simulink model "scheme_L2"  (R2021b)
settings: Solver=ode45  StartTime=0.0  StopTime=10.0  MaxStep=0.001  RelTol=1e-6  AbsTol=1e-8
settings Model: Creator=ALIENWARE  LastModifiedBy=ALIENWARE

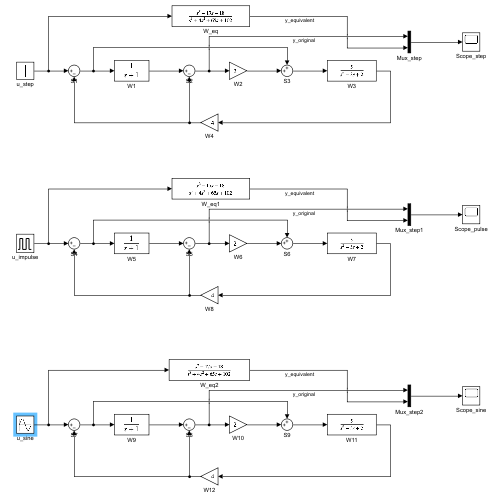
[thumbnail: Simulink's stored preview of the top-level diagram]
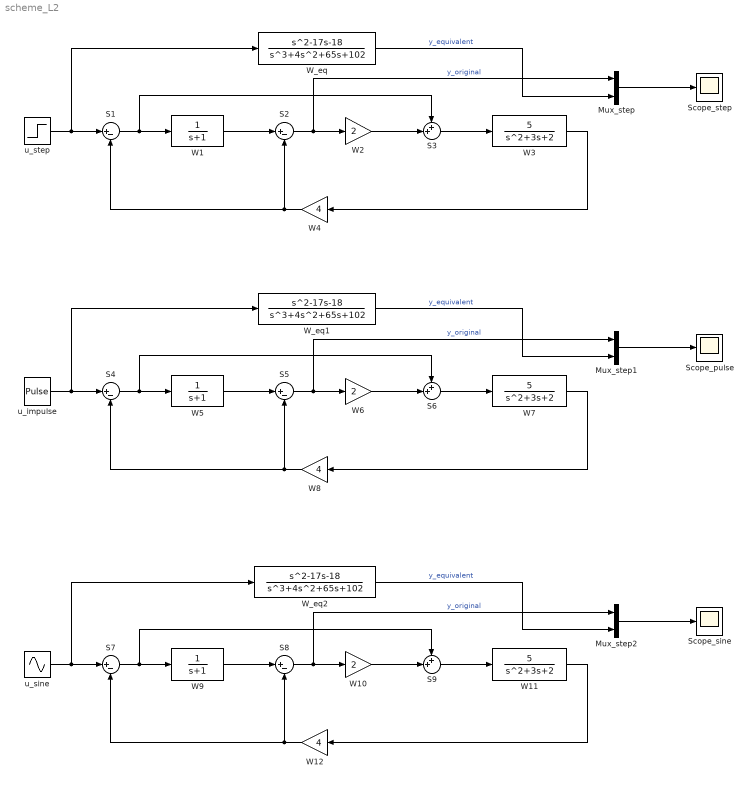
== system scheme_L2 ==
  Mux_step : Mux  Inputs=2
  Mux_step1 : Mux  Inputs=2
  Mux_step2 : Mux  Inputs=2
  S{1..2,4..5,7..8} (6 alike) : Sum  Inputs=|+-
  S3 : Sum  Inputs=++|
  S6 : Sum  Inputs=++|
  S9 : Sum  Inputs=++|
  Scope_pulse : Scope
  Scope_sine : Scope
  Scope_step : Scope
  W1 : TransferFcn  Denominator=[1 1]
  W10 : Gain  Gain=2
  W11 : TransferFcn  Numerator=[5]  Denominator=[1 3 2]
  W12 : Gain  Gain=4
  W2 : Gain  Gain=2
  W3 : TransferFcn  Numerator=[5]  Denominator=[1 3 2]
  W4 : Gain  Gain=4
  W5 : TransferFcn  Denominator=[1 1]
  W6 : Gain  Gain=2
  W7 : TransferFcn  Numerator=[5]  Denominator=[1 3 2]
  W8 : Gain  Gain=4
  W9 : TransferFcn  Denominator=[1 1]
  W_eq : TransferFcn  Numerator=[1 -17 -18]  Denominator=[1 4 65 102]
  W_eq1 : TransferFcn  Numerator=[1 -17 -18]  Denominator=[1 4 65 102]
  W_eq2 : TransferFcn  Numerator=[1 -17 -18]  Denominator=[1 4 65 102]
  u_impulse : DiscretePulseGenerator  PulseType=Time based  Amplitude=100  Period=20  PulseWidth=0.05  PhaseDelay=1
  u_sine : Sin  SampleTime=0
  u_step : Step  SampleTime=0
  wires:
  u_step/1 -> W_eq/1, S1/1
  S1/1 -> S3/1, W1/1
  W1/1 -> S2/1
  S2/1 -> Mux_step/1, W2/1  "y_original"
  W2/1 -> S3/2
  S3/1 -> W3/1
  W3/1 -> W4/1
  W4/1 -> S2/2, S1/2
  W_eq/1 -> Mux_step/2  "y_equivalent"
  Mux_step/1 -> Scope_step/1
  S4/1 -> S6/1, W5/1
  W_eq1/1 -> Mux_step1/2  "y_equivalent"
  W6/1 -> S6/2
  Mux_step1/1 -> Scope_pulse/1
  S5/1 -> Mux_step1/1, W6/1  "y_original"
  W5/1 -> S5/1
  S6/1 -> W7/1
  u_impulse/1 -> W_eq1/1, S4/1
  W8/1 -> S5/2, S4/2
  W7/1 -> W8/1
  S7/1 -> S9/1, W9/1
  W_eq2/1 -> Mux_step2/2  "y_equivalent"
  W10/1 -> S9/2
  Mux_step2/1 -> Scope_sine/1
  S8/1 -> Mux_step2/1, W10/1  "y_original"
  W9/1 -> S8/1
  S9/1 -> W11/1
  u_sine/1 -> W_eq2/1, S7/1
  W12/1 -> S8/2, S7/2
  W11/1 -> W12/1
